simulink model "fft_direct_maptail_test"  (Simulink 7.2)
settings: Solver=VariableStepDiscrete  StartTime=0.0  StopTime=250  RelTol=1e-3
libraries: xbsIndex_r4 x1029, casper_library_misc x88, simulink x2
(part 1 of 9)
settings Model: Creator=User  LastModifiedBy=root
settings OptimizationCC: InitFltsAndDblsToZero=on
settings DebuggingCC: SaveWithDisabledLinksMsg=none  SaveWithParameterizedLinksMsg=none

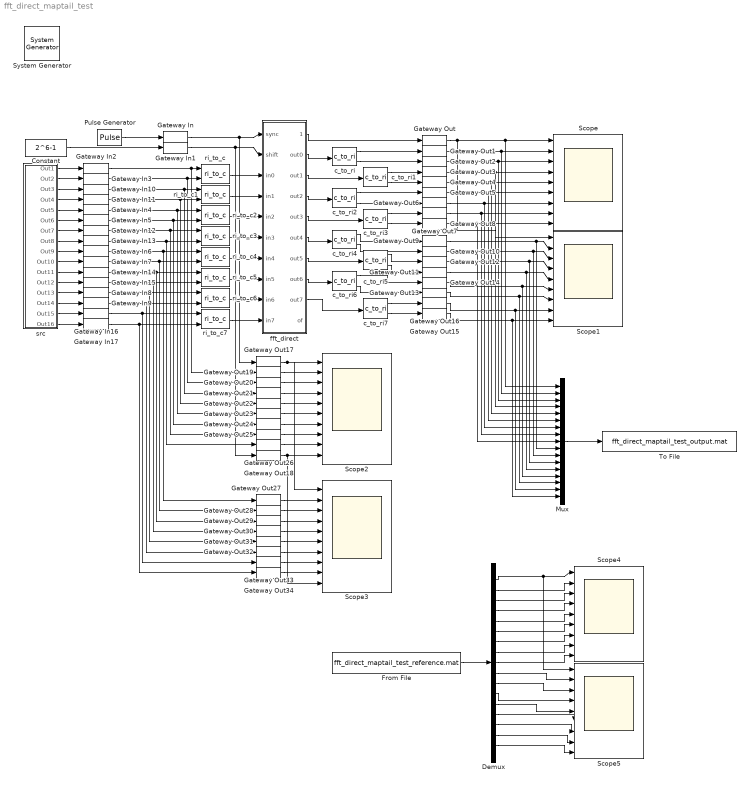
== system fft_direct_maptail_test ==
  " System Generator" : xbsIndex_r4/ System Generator  Tag=genX  SystemSampleTime=-1  xilinxfamily=Virtex4  part=xc4vsx35  speed=-10  package=ff668  synthesis_tool=XST  clock_wrapper=Clock Enables  directory=./netlist  testbench=off  simulink_period=1  sysclk_period=100  dcm_input_clock_period=100  incr_netlist=off  trim_vbits=Everywhere in SubSystem  dbl_ovrd=According to Block Masks  core_generation=According to Block Masks  run_coregen=off  deprecated_control=off  eval_field=0  block_type=sysgen
      settings: block_version=10.1.1
  Constant : Constant  Value=2^6-1  OutDataType=sfix(16)  OutScaling=2^0
  Demux : Demux  Outputs=17
  From File : FromFile  FileName=fft_direct_maptail_test_reference.mat  SampleTime=1
  Gateway In : xbsIndex_r4/Gateway In  arith_type=Boolean  n_bits=16  bin_pt=14  quantization="Round  (unbiased: +/- Inf)"  overflow=Saturate  period=1  dbl_ovrd=off  timing_constraint=None  locs_specified=off  LOCs={}  hdl_port=on  block_type=gatewayin
      settings: infoedit="Gateway in block.  Converts inputs of type Simulink integer, double and fixed point to  Xilinx fixed point type.<P><P>Hardware notes:  In hardware these blocks become top level input ports."  block_version=10.1.1
  Gateway In1 : xbsIndex_r4/Gateway In  arith_type=Unsigned  n_bits=6  bin_pt=0  quantization=Truncate  overflow=Wrap  period=1  dbl_ovrd=off  timing_constraint=None  locs_specified=off  LOCs={}  hdl_port=on  block_type=gatewayin
      settings: infoedit="Gateway in block.  Converts inputs of type Simulink integer, double and fixed point to  Xilinx fixed point type.<P><P>Hardware notes:  In hardware these blocks become top level input ports."  block_version=10.1.1
  Gateway In{2..17} (16 alike) : xbsIndex_r4/Gateway In  arith_type="Signed  (2's comp)"  n_bits=8  bin_pt=7  quantization=Truncate  overflow=Wrap  period=1  dbl_ovrd=off  timing_constraint=None  locs_specified=off  LOCs={}  hdl_port=on  block_type=gatewayin
      settings: infoedit="Gateway in block.  Converts inputs of type Simulink integer, double and fixed point to  Xilinx fixed point type.<P><P>Hardware notes:  In hardware these blocks become top level input ports."  block_version=10.1.1
  Gateway Out{,1..34} (35 alike) : xbsIndex_r4/Gateway Out  hdl_port=on  timing_constraint=None  locs_specified=off  LOCs={}  block_type=gatewayout
      settings: infoedit="Gateway out block.  Converts Xilinx fixed point inputs into ouputs of type Simulink integer, double, or fixed point.<P><P>Hardware notes:  In hardware these blocks become top level output ports or are discarded, depending on how they are configured."  block_version=10.1.1
  Mux : Mux  Inputs=17
  Pulse Generator : DiscretePulseGenerator  Period=2^5  PhaseDelay=13
  Scope{,1,4..5} (4 alike) : Scope  NumInputPorts=9
      Scope settings: YMin=-5~-5~-5~-5~-5~-5~-5~-5~-5  YMax=5~5~5~5~5~5~5~5~5
      Scope1 settings: YMin=-5~-5~-5~-5~-5~-5~-5~-5~-5  YMax=5~5~5~5~5~5~5~5~5
      Scope4 settings: YMin=-5~-5~-5~-5~-5~-5~-5~-5~-5  YMax=5~5~5~5~5~5~5~5~5  SaveName=ScopeData4
      Scope5 settings: YMin=-5~-5~-5~-5~-5~-5~-5~-5~-5  YMax=5~5~5~5~5~5~5~5~5  SaveName=ScopeData5
  Scope2 : Scope  NumInputPorts=10
      settings: YMin=-1~-1~-1~-1~-1~-1~-1~-1~-1~-5  YMax=2~1~1~1~1~1~1~1~1~5  SaveName=ScopeData2
  Scope3 : Scope  NumInputPorts=10
      settings: YMin=-1~-1~-1~-1~-1~-1~-1~-1~-1~-5  YMax=2~1~1~1~1~1~1~1~1~5  SaveName=ScopeData3
  To File : ToFile  Filename=fft_direct_maptail_test_output.mat  MatrixName=output
  c_to_ri{,1..7} (8 alike) : casper_library_misc/c_to_ri  SystemSampleTime=-1  n_bits=16  bin_pt=15
      settings: AttributesFormatString=16_15 r/i
  fft_direct : Subsystem  AncestorBlock=casper_library_ffts/fft_direct  mask(fft_direct){FFTSize=3, input_bit_width=16, coeff_bit_width=16, add_latency=2, mult_latency=2, bram_latency=2, conv_latency=2, quantization=Truncate, overflow=Wrap, map_tail=on, LargerFFTSize=5, StartStage=3, arch=Virtex5, opt_target=logic, coeffs_bit_limit=8, specify_mult=off, mult_spec=[2                                      2], dsp48_adders=off}
      mask prompts: FFTSize "Size of FFT: (2^?)"; input_bit_width "Input/Output Bit Width"; coeff_bit_width "Coefficient Bit Width"; add_latency "Add Latency"; mult_latency "Mult Latency"; bram_latency "BRAM Latency"; conv_latency "Convert latency"; quantization "Quantization Behavior"; overflow "Overflow Behavior"; map_tail "Map Tail of Larger FFT"; LargerFFTSize "Size of Larger FFT (2^?):"; StartStage "Start Stage of Map Tail:"; arch "Architecture"; opt_target "Use less"; coeffs_bit_limit "Number bits above which to store stage's coefficients in BRAM (2^? bits)"; specify_mult "Specify multiplier use (behavioural HDL if not specified)"; mult_spec "Multiplier specification (0=core, 1=behavioural HDL, 2=embedded) (left=1st stage)"; dsp48_adders "DSP48 adders in butterfly"
      mask help:
      | Implements an N-point FFT with the classic
      | butterfly structure with N inputs and N outputs
      mask init:
      | fft_direct_init(gcb,...
      |     'FFTSize', FFTSize, ...
      |     'input_bit_width', input_bit_width, ...
      |     'coeff_bit_width', coeff_bit_width, ...
      |     'add_latency', add_latency, ...
      |     'mult_latency', mult_latency, ...
      |     'bram_latency', bram_latency, ...
      |     'conv_latency', conv_latency, ...
      |     'quantization', quantization, ...
      |     'overflow', overflow, ...
      |     'map_tail', map_tail, ...
      |     'LargerFFTSize', LargerFFTSize, ...
      |     'StartStage', StartStage, ...
      |     'arch', arch, ...
      |     'opt_target', opt_target, ...
      |     'coeffs_bit_limit', coeffs_bit_limit, ...
      |     'specify_mult', specify_mult, ...
      |     'mult_spec', mult_spec, ...
      |     'dsp48_adders', dsp48_adders);
      settings: AttributesFormatString=|
      | Virtex5
      | stages [3  4  5] of 5
      | [16,16]
      | Truncate
      | Wrap
      mask StyleString: edit,edit,edit,edit,edit,edit,edit,popup(Truncate|Round  (unbiased: +/- Inf)|Round  (unbiased: Even Values)),popup(Wrap|Saturate|Error),checkbox,edit,edit,popup(Virtex2Pro|Virtex5),popup(logic|multipliers),edit,checkbox,edit,checkbox
      mask CallbackString:
      | % fft_size = eval(get_param(gcb, 'FFTSize'));
      | % old_vec = eval(get_param(gcb, 'mult_spec'));
      | 
      | % vec = 2.*ones(1,fft_size);
      | % old_size = length(old_vec);
      | 
      | % if(old_size <= fft_size),
      | %     size = old_size;
      | % else,
      | %     size = fft_size;
      | % end
      | 
      | % for n = 1:size, vec(n) = old_vec(n); end
      | % set_param(gcb, 'mult_spec', mat2str(vec));|||||||||map_tail = get_param(gcb,'map_tail');
      | visibs = get_param(gcb, 'MaskVisibilities');
      | if( strcmp(map_tail,'off')),
      |     visibs{11} = 'off';
      |     visibs{12} = 'off';
      | else,
      |     visibs{11} = 'on';
      |     visibs{12} = 'on';
      | end
      | set_param(gcb, 'MaskVisibilities', visibs);
      | |||fft_callback_arch(gcb);|||specify_mult = get_param(gcb,'specify_mult');
      | visibs = get_param(gcb, 'MaskVisibilities');
      | if( strcmp(specify_mult,'off')), visibs{17} = 'off';
      | else, visibs{17} = 'on';
      | end
      | set_param(gcb, 'MaskVisibilities', visibs);
      | |% vec = eval( get_param(gcb, 'mult_spec'));
      | % vec_size = length(vec);
      | % fft_size = eval( get_param(gcb, 'FFTSize'));
      | % new_vec = 2.*ones(1, fft_size);
      | 
      | % if(vec_size <= fft_size), size = vec_size;
      | % else size = fft_size;
      | % end
      | 
      | % for n=1:size
      | %     new_vec(n) = vec(n);
      | % end
      | % set_param(gcb, 'mult_spec', mat2str(new_vec));|fft_callback_dsp48_adders(gcb);
  ri_to_c{,1..7} (8 alike) : casper_library_misc/ri_to_c  SystemSampleTime=-1
  src : Subsystem
  wires:
  Pulse Generator/1 -> Gateway In/1
  Gateway In/1 -> Gateway Out17/1, fft_direct/1(sync)
  Constant/1 -> Gateway In1/1
  Gateway In1/1 -> Gateway Out18/1, fft_direct/2(shift)
  fft_direct/2(out0) -> c_to_ri/1
  fft_direct/1(sync_out) -> Gateway Out/1
  c_to_ri/1 -> Gateway Out1/1
  c_to_ri/2 -> Gateway Out2/1
  fft_direct/3(out1) -> c_to_ri1/1
  c_to_ri1/1 -> Gateway Out3/1
  c_to_ri1/2 -> Gateway Out4/1
  Gateway Out/1 -> Scope1/1, Scope/1, Mux/1
  Gateway Out1/1 -> Scope/2, Mux/2
  Gateway Out2/1 -> Scope/3, Mux/3
  Gateway Out3/1 -> Scope/4, Mux/4
  Gateway Out4/1 -> Scope/5, Mux/5
  fft_direct/4(out2) -> c_to_ri2/1
  c_to_ri2/1 -> Gateway Out5/1
  c_to_ri2/2 -> Gateway Out6/1
  fft_direct/5(out3) -> c_to_ri3/1
  c_to_ri3/1 -> Gateway Out7/1
  c_to_ri3/2 -> Gateway Out8/1
  c_to_ri4/1 -> Gateway Out9/1
  c_to_ri4/2 -> Gateway Out10/1
  c_to_ri5/1 -> Gateway Out12/1
  c_to_ri5/2 -> Gateway Out11/1
  c_to_ri6/1 -> Gateway Out14/1
  c_to_ri6/2 -> Gateway Out13/1
  c_to_ri7/1 -> Gateway Out16/1
  c_to_ri7/2 -> Gateway Out15/1
  fft_direct/6(out4) -> c_to_ri4/1
  fft_direct/7(out5) -> c_to_ri5/1
  fft_direct/8(out6) -> c_to_ri6/1
  fft_direct/9(out7) -> c_to_ri7/1
  Gateway Out5/1 -> Scope/6, Mux/6
  Gateway Out6/1 -> Scope/7, Mux/7
  Gateway Out7/1 -> Scope/8, Mux/8
  Gateway Out8/1 -> Scope/9, Mux/9
  Gateway Out9/1 -> Scope1/2, Mux/10
  Gateway Out10/1 -> Scope1/3, Mux/11
  Gateway Out12/1 -> Scope1/4, Mux/12
  Gateway Out11/1 -> Scope1/5, Mux/13
  Gateway Out14/1 -> Scope1/6, Mux/14
  Gateway Out13/1 -> Scope1/7, Mux/15
  Gateway Out16/1 -> Scope1/8, Mux/16
  Gateway Out15/1 -> Scope1/9, Mux/17
  Mux/1 -> To File/1
  Gateway In2/1 -> ri_to_c/1, Gateway Out19/1
  Gateway In3/1 -> ri_to_c/2, Gateway Out20/1
  Gateway In10/1 -> ri_to_c1/1, Gateway Out21/1
  Gateway In11/1 -> ri_to_c1/2, Gateway Out22/1
  Gateway In4/1 -> ri_to_c2/1, Gateway Out23/1
  Gateway In5/1 -> ri_to_c2/2, Gateway Out24/1
  Gateway In12/1 -> ri_to_c3/1, Gateway Out25/1
  Gateway In13/1 -> ri_to_c3/2, Gateway Out26/1
  Gateway In6/1 -> ri_to_c4/1, Gateway Out27/1
  Gateway In7/1 -> ri_to_c4/2, Gateway Out28/1
  Gateway In8/1 -> ri_to_c6/1, Gateway Out31/1
  Gateway In9/1 -> ri_to_c6/2, Gateway Out32/1
  Gateway In14/1 -> ri_to_c5/1, Gateway Out29/1
  Gateway In15/1 -> ri_to_c5/2, Gateway Out30/1
  src/1(Out1) -> Gateway In2/1
  src/2(Out2) -> Gateway In3/1
  src/3(Out3) -> Gateway In10/1
  src/4(Out4) -> Gateway In11/1
  src/5(Out5) -> Gateway In4/1
  src/6(Out6) -> Gateway In5/1
  src/7(Out7) -> Gateway In12/1
  src/8(Out8) -> Gateway In13/1
  src/9(Out9) -> Gateway In6/1
  src/10(Out10) -> Gateway In7/1
  src/11(Out11) -> Gateway In14/1
  src/12(Out12) -> Gateway In15/1
  src/13(Out13) -> Gateway In8/1
  src/14(Out14) -> Gateway In9/1
  Gateway In17/1 -> ri_to_c7/2, Gateway Out34/1
  src/15(Out15) -> Gateway In16/1
  src/16(Out16) -> Gateway In17/1
  Gateway In16/1 -> ri_to_c7/1, Gateway Out33/1
  ri_to_c/1 -> fft_direct/3(in0)
  ri_to_c1/1 -> fft_direct/4(in1)
  ri_to_c2/1 -> fft_direct/5(in2)
  ri_to_c3/1 -> fft_direct/6(in3)
  ri_to_c4/1 -> fft_direct/7(in4)
  ri_to_c5/1 -> fft_direct/8(in5)
  ri_to_c6/1 -> fft_direct/9(in6)
  ri_to_c7/1 -> fft_direct/10(in7)
  Gateway Out18/1 -> Scope2/10, Scope3/10
  Gateway Out17/1 -> Scope2/1, Scope3/1
  Gateway Out19/1 -> Scope2/2
  Gateway Out20/1 -> Scope2/3
  Gateway Out21/1 -> Scope2/4
  Gateway Out22/1 -> Scope2/5
  Gateway Out23/1 -> Scope2/6
  Gateway Out24/1 -> Scope2/7
  Gateway Out25/1 -> Scope2/8
  Gateway Out26/1 -> Scope2/9
  Gateway Out27/1 -> Scope3/2
  Gateway Out28/1 -> Scope3/3
  Gateway Out29/1 -> Scope3/4
  Gateway Out30/1 -> Scope3/5
  Gateway Out31/1 -> Scope3/6
  Gateway Out32/1 -> Scope3/7
  Gateway Out33/1 -> Scope3/8
  Gateway Out34/1 -> Scope3/9
  From File/1 -> Demux/1
  Demux/1 -> Scope4/1, Scope5/1
  Demux/2 -> Scope4/2
  Demux/3 -> Scope4/3
  Demux/4 -> Scope4/4
  Demux/5 -> Scope4/5
  Demux/6 -> Scope4/6
  Demux/7 -> Scope4/7
  Demux/8 -> Scope4/8
  Demux/9 -> Scope4/9
  Demux/10 -> Scope5/2
  Demux/11 -> Scope5/3
  Demux/12 -> Scope5/4
  Demux/13 -> Scope5/5
  Demux/14 -> Scope5/6
  Demux/15 -> Scope5/7
  Demux/16 -> Scope5/8
  Demux/17 -> Scope5/9
